simulink library "mssSimulink"  (R2024a)
settings: Solver=ode45  StartTime=0.0  StopTime=10.0  RelTol=1e-3
undefined symbols (not defined in the file): ABC, CN_data, CX_data, CY_data, D, G, Hoerner, K_supply, kt2ms, MA, magnitude, MRB, pathlength, RAO_Amp, RAO_Dir, RAO_Freq, RAO_Phase, RAO_Vel, RAO_yaw_back, RAO_yaw_quant, RAO_yaw_quantization_flag, rho_a, slcm, T_supply, table, vessel, vesselABC
libraries: $bdroot x99, simulink x13
(part 8 of 9)

== system mssSimulink/Guidance/Waypoint guidance block/vs_calculations/vs_theta_calc ==
  xd_theta : Inport
  xd_theta_2 : Inport  Port=2
  yd_theta : Inport  Port=3
  yd_theta_2 : Inport  Port=4
  ud : Inport  Port=5
  Fcn1 : Fcn  Expr=u^(3/2)
  Gain1 : Gain  Gain=-1  SaturateOnIntegerOverflow=on  OutDataTypeStr=Inherit: Same as input  ParamDataTypeStr=Inherit: Same as input
  Math Function2 : Math  Operator=square  SignedPower=on
  Math Function3 : Math  Operator=square  SignedPower=on
  Product4 : Product  InputSameDT=on  SaturateOnIntegerOverflow=on  OutDataTypeStr=Inherit: Same as first input
  Product5 : Product  InputSameDT=on  SaturateOnIntegerOverflow=on  OutDataTypeStr=Inherit: Same as first input
  Product6 : Product  Inputs=/*  InputSameDT=on  SaturateOnIntegerOverflow=on  OutDataTypeStr=Inherit: Same as first input
  Product7 : Product  InputSameDT=on  SaturateOnIntegerOverflow=on  OutDataTypeStr=Inherit: Same as first input
  Sum2 : Sum  Inputs=|++  InputSameDT=on  SaturateOnIntegerOverflow=on  OutDataTypeStr=Inherit: Same as first input
  Sum3 : Sum  Inputs=|++  InputSameDT=on  SaturateOnIntegerOverflow=on  OutDataTypeStr=Inherit: Same as first input
  vs_theta : Outport  VectorParamsAs1DForOutWhenUnconnected=off
  wires:
  xd_theta/1 -> Math Function2/1, Product4/1
  yd_theta/1 -> Math Function3/1, Product5/1
  Math Function2/1 -> Sum2/1
  Math Function3/1 -> Sum2/2
  Sum2/1 -> Fcn1/1
  xd_theta_2/1 -> Product4/2
  yd_theta_2/1 -> Product5/2
  Product4/1 -> Sum3/1
  Product5/1 -> Sum3/2
  Fcn1/1 -> Product6/1
  Sum3/1 -> Product6/2
  Product6/1 -> Gain1/1
  Gain1/1 -> Product7/1
  ud/1 -> Product7/2
  Product7/1 -> vs_theta/1

== system mssSimulink/Hydrodynamics/6-DOF maneuvering model (unified model with fluid memory)/Model Info1/EmptySubsystem ==

== system mssSimulink/Hydrodynamics/Cross-flow drag and surge resistance/Cross-flow drag trapezoidal integration/multiply with 0.5 ==
  In1 : Inport
  Action Port : ActionPort  InitializeStates=reset
  Gain : Gain  Gain=0.5
  Out1 : Outport
  wires:
  In1/1 -> Gain/1
  Gain/1 -> Out1/1

== system mssSimulink/Hydrodynamics/Cross-flow drag and surge resistance/Cross-flow drag trapezoidal integration/multiply with 1 ==
  In1 : Inport
  Action Port : ActionPort  InitializeStates=reset
  Out1 : Outport
  wires:
  In1/1 -> Out1/1

== system mssSimulink/Hydrodynamics/WD for heading1/Wave component loop/WD RAO tables ==
  beta : Inport
  w : Inport  Port=2
  U : Inport  Port=3
  Constant : Constant  Value=0
  Lookup Table (n-D) Wavedrift 1 : Lookup_n-D  NumberOfTableDimensions=3  BreakpointsForDimension1=WD_Freq  BreakpointsForDimension2=vessel.headings  BreakpointsForDimension3=RAO_Vel  IndexSearchMethod=Linear search  BeginIndexSearchUsingPreviousIndexResult=on  Table=WD_Amp{1}  ExtrapMethod=Clip  DiagnosticForOutOfRangeInput=Warning  InternalRulePriority=Speed  RndMeth=Simplest
      settings: InputPortMap=u0,u1,u2
  Lookup Table (n-D) Wavedrift 2 : Lookup_n-D  NumberOfTableDimensions=3  BreakpointsForDimension1=WD_Freq  BreakpointsForDimension2=vessel.headings  BreakpointsForDimension3=RAO_Vel  IndexSearchMethod=Linear search  BeginIndexSearchUsingPreviousIndexResult=on  Table=WD_Amp{2}  ExtrapMethod=Clip  DiagnosticForOutOfRangeInput=Warning  InternalRulePriority=Speed  RndMeth=Simplest
      settings: InputPortMap=u0,u1,u2
  Lookup Table (n-D) Wavedrift 3 : Lookup_n-D  NumberOfTableDimensions=3  BreakpointsForDimension1=WD_Freq  BreakpointsForDimension2=vessel.headings  BreakpointsForDimension3=RAO_Vel  IndexSearchMethod=Linear search  BeginIndexSearchUsingPreviousIndexResult=on  Table=WD_Amp{3}  ExtrapMethod=Clip  DiagnosticForOutOfRangeInput=Warning  InternalRulePriority=Speed  RndMeth=Simplest
      settings: InputPortMap=u0,u1,u2
  Mux1 : Mux  Inputs=6
  amp : Outport
  wires:
  Mux1/1 -> amp/1
  Lookup Table (n-D) Wavedrift 3/1 -> Mux1/6
  Lookup Table (n-D) Wavedrift 2/1 -> Mux1/2
  Lookup Table (n-D) Wavedrift 1/1 -> Mux1/1
  U/1 -> Lookup Table (n-D) Wavedrift 2/3, Lookup Table (n-D) Wavedrift 3/3, Lookup Table (n-D) Wavedrift 1/3
  beta/1 -> Lookup Table (n-D) Wavedrift 2/2, Lookup Table (n-D) Wavedrift 3/2, Lookup Table (n-D) Wavedrift 1/2
  Constant/1 -> Mux1/3, Mux1/4, Mux1/5
  w/1 -> Lookup Table (n-D) Wavedrift 2/1, Lookup Table (n-D) Wavedrift 3/1, Lookup Table (n-D) Wavedrift 1/1

== system mssSimulink/Hydrodynamics/WD for heading1/Wave component loop/[-pi pi] to [0 2pi] ==
  note: x
  x [-pi pi] : Inport
  Constant : Constant  Value=2*pi
  Constant1 : Constant  Value=0
  Sign : Signum
  Sum : Sum  Inputs=|++  SaturateOnIntegerOverflow=on
  Switch : Switch  SaturateOnIntegerOverflow=off  InputSameDT=off
  0<y<2pi : Outport
  wires:
  x [-pi pi]/1 -> Sign/1, Sum/2
  Switch/1 -> Sum/1
  Sum/1 -> 0<y<2pi/1
  Sign/1 -> Switch/2
  Constant/1 -> Switch/3
  Constant1/1 -> Switch/1

== system mssSimulink/Hydrodynamics/Wave loads (U>0)/Wave loads U = U1/psi1 ==
  k : Inport
  0 or 1 : Inport  Port=2
  Gain1 : Gain  Gain=20
  Gain2 : Gain  Gain=10
  Product : Product  RndMeth=Zero
  Sum7 : Sum  Inputs=-+|
  Sum8 : Sum  Inputs=++|
  const : Constant  Value=18
  psi : Outport
  wires:
  0 or 1/1 -> Product/2
  Sum8/1 -> psi/1
  k/1 -> Gain2/1, Sum7/1
  Gain2/1 -> Sum8/1
  Product/1 -> Sum8/2
  Gain1/1 -> Product/1
  Sum7/1 -> Gain1/1
  const/1 -> Sum7/2

== system mssSimulink/Hydrodynamics/Wave loads (U>0)/Wave loads U = U1/psi2 ==
  k : Inport
  0 or 1 : Inport  Port=2
  Gain1 : Gain  Gain=20
  Gain2 : Gain  Gain=10
  Product : Product  RndMeth=Zero
  Sum7 : Sum  Inputs=-+|
  Sum8 : Sum  Inputs=++|
  const : Constant  Value=18
  psi : Outport
  wires:
  0 or 1/1 -> Product/2
  Sum8/1 -> psi/1
  k/1 -> Gain2/1, Sum7/1
  Gain2/1 -> Sum8/1
  Product/1 -> Sum8/2
  Gain1/1 -> Product/1
  Sum7/1 -> Gain1/1
  const/1 -> Sum7/2

== system mssSimulink/Hydrodynamics/Wave loads (U>0)/Wave loads U = U2/Wave loads for heading1 ==
  eta : Inport
  psi : Inport  Port=2
  psi_wave : Inport  Port=3
  wavenum : Inport  Port=4
  Omega : Inport  Port=5
  Phase : Inport  Port=6
  Zeta_a : Inport  Port=7
  U_idx : Inport  Port=8
  Clock : Clock
  "Position phase " : $bdroot/Modelling/Environmental Loads/Utilities/Position phase
  Product1 : Product  Inputs=**  SaturateOnIntegerOverflow=on  OutDataTypeStr=Inherit: Same as first input
  Sum : Sum  Inputs=-++  SaturateOnIntegerOverflow=on
  Sum1 : Sum  Inputs=-+|
  Wave component loop : Subsystem  TreatAsAtomicUnit=on
  Width : Width  DataType=int32
  tau_WF : Outport
  tau_WD : Outport  Port=2
  wires:
  psi/1 -> Sum1/1  "psi"
  U_idx/1 -> Wave component loop/6(U_idx)
  Wave component loop/2(tau_WD) -> tau_WD/1
  Sum1/1 -> Wave component loop/2(Psi_r)
  Zeta_a/1 -> Wave component loop/5(Zeta_a)
  Phase/1 -> Sum/3
  Omega/1 -> Width/1, Wave component loop/3(Omega), Product1/1
  wavenum/1 -> "Position phase "/2
  psi_wave/1 -> Sum1/2, "Position phase "/1
  eta/1 -> "Position phase "/3
  Wave component loop/1(tau_WF) -> tau_WF/1
  Product1/1 -> Sum/2
  Clock/1 -> Product1/2
  Sum/1 -> Wave component loop/4(Phase_tot)  "Phase_tot"
  Width/1 -> Wave component loop/1(number of iterations)
  "Position phase "/1 -> Sum/1

== system mssSimulink/Hydrodynamics/Wave loads (U>0)/Wave loads U = U2/Wave loads for heading2 ==
  eta : Inport
  psi : Inport  Port=2
  psi_wave : Inport  Port=3
  wavenum : Inport  Port=4
  Omega : Inport  Port=5
  Phase : Inport  Port=6
  Zeta_a : Inport  Port=7
  U : Inport  Port=8
  Clock : Clock
  "Position phase " : $bdroot/Modelling/Environmental Loads/Utilities/Position phase
  Product1 : Product  Inputs=**  SaturateOnIntegerOverflow=on  OutDataTypeStr=Inherit: Same as first input
  Sum : Sum  Inputs=-++  SaturateOnIntegerOverflow=on
  Sum1 : Sum  Inputs=-+|
  Wave component loop : Subsystem  TreatAsAtomicUnit=on
  Width : Width  DataType=int32
  tau_WF : Outport
  tau_WD : Outport  Port=2
  wires:
  psi/1 -> Sum1/1  "psi"
  U/1 -> Wave component loop/6(U)
  Wave component loop/2(tau_WD) -> tau_WD/1
  Sum1/1 -> Wave component loop/2(Psi_r)
  Zeta_a/1 -> Wave component loop/5(Zeta_a)
  Phase/1 -> Sum/3
  Omega/1 -> Width/1, Wave component loop/3(Omega), Product1/1
  wavenum/1 -> "Position phase "/2
  psi_wave/1 -> Sum1/2, "Position phase "/1
  eta/1 -> "Position phase "/3
  Wave component loop/1(tau_WF) -> tau_WF/1
  Product1/1 -> Sum/2
  Clock/1 -> Product1/2
  Sum/1 -> Wave component loop/4(Phase_tot)  "Phase_tot"
  Width/1 -> Wave component loop/1(number of iterations)
  "Position phase "/1 -> Sum/1

== system mssSimulink/Hydrodynamics/Wave loads (U>0)/Wave loads U = U2/psi1 ==
  k : Inport
  0 or 1 : Inport  Port=2
  Gain1 : Gain  Gain=20
  Gain2 : Gain  Gain=10
  Product : Product  RndMeth=Zero
  Sum7 : Sum  Inputs=-+|
  Sum8 : Sum  Inputs=++|
  const : Constant  Value=18
  psi : Outport
  wires:
  0 or 1/1 -> Product/2
  Sum8/1 -> psi/1
  k/1 -> Gain2/1, Sum7/1
  Gain2/1 -> Sum8/1
  Product/1 -> Sum8/2
  Gain1/1 -> Product/1
  Sum7/1 -> Gain1/1
  const/1 -> Sum7/2

== system mssSimulink/Hydrodynamics/Wave loads (U>0)/Wave loads U = U2/psi2 ==
  k : Inport
  0 or 1 : Inport  Port=2
  Gain1 : Gain  Gain=20
  Gain2 : Gain  Gain=10
  Product : Product  RndMeth=Zero
  Sum7 : Sum  Inputs=-+|
  Sum8 : Sum  Inputs=++|
  const : Constant  Value=18
  psi : Outport
  wires:
  0 or 1/1 -> Product/2
  Sum8/1 -> psi/1
  k/1 -> Gain2/1, Sum7/1
  Gain2/1 -> Sum8/1
  Product/1 -> Sum8/2
  Gain1/1 -> Product/1
  Sum7/1 -> Gain1/1
  const/1 -> Sum7/2

== system mssSimulink/Hydrodynamics/Wave loads for heading1/Wave component loop/Force RAO tables ==
  beta : Inport
  w : Inport  Port=2
  U : Inport  Port=3
  Lookup Table (n-D) Amp1 : Lookup_n-D  NumberOfTableDimensions=3  BreakpointsForDimension1=ForceRAO_Freq  BreakpointsForDimension2=vessel.headings  BreakpointsForDimension3=RAO_Vel  IndexSearchMethod=Linear search  BeginIndexSearchUsingPreviousIndexResult=on  Table=ForceRAO_Amp{1}  ExtrapMethod=Clip  DiagnosticForOutOfRangeInput=Warning  InternalRulePriority=Speed  RndMeth=Simplest
      settings: InputPortMap=u0,u1,u2
  Lookup Table (n-D) Amp2 : Lookup_n-D  NumberOfTableDimensions=3  BreakpointsForDimension1=ForceRAO_Freq  BreakpointsForDimension2=vessel.headings  BreakpointsForDimension3=RAO_Vel  IndexSearchMethod=Linear search  BeginIndexSearchUsingPreviousIndexResult=on  Table=ForceRAO_Amp{2}  ExtrapMethod=Clip  DiagnosticForOutOfRangeInput=Warning  InternalRulePriority=Speed  RndMeth=Simplest
      settings: InputPortMap=u0,u1,u2
  Lookup Table (n-D) Amp3 : Lookup_n-D  NumberOfTableDimensions=3  BreakpointsForDimension1=ForceRAO_Freq  BreakpointsForDimension2=vessel.headings  BreakpointsForDimension3=RAO_Vel  IndexSearchMethod=Linear search  BeginIndexSearchUsingPreviousIndexResult=on  Table=ForceRAO_Amp{3}  ExtrapMethod=Clip  DiagnosticForOutOfRangeInput=Warning  InternalRulePriority=Speed  RndMeth=Simplest
      settings: InputPortMap=u0,u1,u2
  Lookup Table (n-D) Amp4 : Lookup_n-D  NumberOfTableDimensions=3  BreakpointsForDimension1=ForceRAO_Freq  BreakpointsForDimension2=vessel.headings  BreakpointsForDimension3=RAO_Vel  IndexSearchMethod=Linear search  BeginIndexSearchUsingPreviousIndexResult=on  Table=ForceRAO_Amp{4}  ExtrapMethod=Clip  DiagnosticForOutOfRangeInput=Warning  InternalRulePriority=Speed  RndMeth=Simplest
      settings: InputPortMap=u0,u1,u2
  Lookup Table (n-D) Amp5 : Lookup_n-D  NumberOfTableDimensions=3  BreakpointsForDimension1=ForceRAO_Freq  BreakpointsForDimension2=vessel.headings  BreakpointsForDimension3=RAO_Vel  IndexSearchMethod=Linear search  BeginIndexSearchUsingPreviousIndexResult=on  Table=ForceRAO_Amp{5}  ExtrapMethod=Clip  DiagnosticForOutOfRangeInput=Warning  InternalRulePriority=Speed  RndMeth=Simplest
      settings: InputPortMap=u0,u1,u2
  Lookup Table (n-D) Amp6 : Lookup_n-D  NumberOfTableDimensions=3  BreakpointsForDimension1=ForceRAO_Freq  BreakpointsForDimension2=vessel.headings  BreakpointsForDimension3=RAO_Vel  IndexSearchMethod=Linear search  BeginIndexSearchUsingPreviousIndexResult=on  Table=ForceRAO_Amp{6}  ExtrapMethod=Clip  DiagnosticForOutOfRangeInput=Warning  InternalRulePriority=Speed  RndMeth=Simplest
      settings: InputPortMap=u0,u1,u2
  Lookup Table (n-D) Phase : Lookup_n-D  NumberOfTableDimensions=3  BreakpointsForDimension1=ForceRAO_Freq  BreakpointsForDimension2=vessel.headings  BreakpointsForDimension3=RAO_Vel  IndexSearchMethod=Linear search  BeginIndexSearchUsingPreviousIndexResult=on  Table=ForceRAO_Phase{3}  ExtrapMethod=Clip  DiagnosticForOutOfRangeInput=Warning  InternalRulePriority=Speed  RndMeth=Simplest
      settings: InputPortMap=u0,u1,u2
  Lookup Table (n-D) Phase1 : Lookup_n-D  NumberOfTableDimensions=3  BreakpointsForDimension1=ForceRAO_Freq  BreakpointsForDimension2=vessel.headings  BreakpointsForDimension3=RAO_Vel  IndexSearchMethod=Linear search  BeginIndexSearchUsingPreviousIndexResult=on  Table=ForceRAO_Phase{1}  ExtrapMethod=Clip  DiagnosticForOutOfRangeInput=Warning  InternalRulePriority=Speed  RndMeth=Simplest
      settings: InputPortMap=u0,u1,u2
  Lookup Table (n-D) Phase2 : Lookup_n-D  NumberOfTableDimensions=3  BreakpointsForDimension1=ForceRAO_Freq  BreakpointsForDimension2=vessel.headings  BreakpointsForDimension3=RAO_Vel  IndexSearchMethod=Linear search  BeginIndexSearchUsingPreviousIndexResult=on  Table=ForceRAO_Phase{2}  ExtrapMethod=Clip  DiagnosticForOutOfRangeInput=Warning  InternalRulePriority=Speed  RndMeth=Simplest
      settings: InputPortMap=u0,u1,u2
  Lookup Table (n-D) Phase4 : Lookup_n-D  NumberOfTableDimensions=3  BreakpointsForDimension1=ForceRAO_Freq  BreakpointsForDimension2=vessel.headings  BreakpointsForDimension3=RAO_Vel  IndexSearchMethod=Linear search  BeginIndexSearchUsingPreviousIndexResult=on  Table=ForceRAO_Phase{4}  ExtrapMethod=Clip  DiagnosticForOutOfRangeInput=Warning  InternalRulePriority=Speed  RndMeth=Simplest
      settings: InputPortMap=u0,u1,u2
  Lookup Table (n-D) Phase5 : Lookup_n-D  NumberOfTableDimensions=3  BreakpointsForDimension1=ForceRAO_Freq  BreakpointsForDimension2=vessel.headings  BreakpointsForDimension3=RAO_Vel  IndexSearchMethod=Linear search  BeginIndexSearchUsingPreviousIndexResult=on  Table=ForceRAO_Phase{5}  ExtrapMethod=Clip  DiagnosticForOutOfRangeInput=Warning  InternalRulePriority=Speed  RndMeth=Simplest
      settings: InputPortMap=u0,u1,u2
  Lookup Table (n-D) Phase6 : Lookup_n-D  NumberOfTableDimensions=3  BreakpointsForDimension1=ForceRAO_Freq  BreakpointsForDimension2=vessel.headings  BreakpointsForDimension3=RAO_Vel  IndexSearchMethod=Linear search  BeginIndexSearchUsingPreviousIndexResult=on  Table=ForceRAO_Phase{6}  ExtrapMethod=Clip  DiagnosticForOutOfRangeInput=Warning  InternalRulePriority=Speed  RndMeth=Simplest
      settings: InputPortMap=u0,u1,u2
  Mux1 : Mux  Inputs=6
  Mux2 : Mux  Inputs=6
  amp : Outport
  phase : Outport  Port=2
  wires:
  w/1 -> Lookup Table (n-D) Amp1/1, Lookup Table (n-D) Amp2/1, Lookup Table (n-D) Amp3/1, Lookup Table (n-D) Amp4/1, Lookup Table (n-D) Amp5/1, Lookup Table (n-D) Amp6/1, Lookup Table (n-D) Phase1/1, Lookup Table (n-D) Phase2/1, Lookup Table (n-D) Phase/1, Lookup Table (n-D) Phase4/1, Lookup Table (n-D) Phase6/1, Lookup Table (n-D) Phase5/1
  Lookup Table (n-D) Phase5/1 -> Mux2/5
  Lookup Table (n-D) Phase/1 -> Mux2/3
  Lookup Table (n-D) Phase1/1 -> Mux2/1
  beta/1 -> Lookup Table (n-D) Amp1/2, Lookup Table (n-D) Amp2/2, Lookup Table (n-D) Amp3/2, Lookup Table (n-D) Amp4/2, Lookup Table (n-D) Amp5/2, Lookup Table (n-D) Amp6/2, Lookup Table (n-D) Phase1/2, Lookup Table (n-D) Phase2/2, Lookup Table (n-D) Phase/2, Lookup Table (n-D) Phase4/2, Lookup Table (n-D) Phase6/2, Lookup Table (n-D) Phase5/2
  Lookup Table (n-D) Phase4/1 -> Mux2/4
  Lookup Table (n-D) Phase2/1 -> Mux2/2
  Lookup Table (n-D) Phase6/1 -> Mux2/6
  Lookup Table (n-D) Amp4/1 -> Mux1/4
  U/1 -> Lookup Table (n-D) Amp1/3, Lookup Table (n-D) Amp2/3, Lookup Table (n-D) Amp3/3, Lookup Table (n-D) Amp4/3, Lookup Table (n-D) Amp5/3, Lookup Table (n-D) Amp6/3, Lookup Table (n-D) Phase1/3, Lookup Table (n-D) Phase2/3, Lookup Table (n-D) Phase/3, Lookup Table (n-D) Phase4/3, Lookup Table (n-D) Phase6/3, Lookup Table (n-D) Phase5/3
  Lookup Table (n-D) Amp1/1 -> Mux1/1
  Lookup Table (n-D) Amp3/1 -> Mux1/3
  Lookup Table (n-D) Amp5/1 -> Mux1/5
  Lookup Table (n-D) Amp2/1 -> Mux1/2
  Lookup Table (n-D) Amp6/1 -> Mux1/6
  Mux2/1 -> phase/1
  Mux1/1 -> amp/1

== system mssSimulink/Hydrodynamics/Wave loads for heading1/Wave component loop/WD RAO tables ==
  beta : Inport
  w : Inport  Port=2
  U : Inport  Port=3
  Constant : Constant  Value=0
  Lookup Table (n-D) Wavedrift 1 : Lookup_n-D  NumberOfTableDimensions=3  BreakpointsForDimension1=WD_Freq  BreakpointsForDimension2=vessel.headings  BreakpointsForDimension3=RAO_Vel  IndexSearchMethod=Linear search  BeginIndexSearchUsingPreviousIndexResult=on  Table=WD_Amp{1}  ExtrapMethod=Clip  DiagnosticForOutOfRangeInput=Warning  InternalRulePriority=Speed  RndMeth=Simplest
      settings: InputPortMap=u0,u1,u2
  Lookup Table (n-D) Wavedrift 2 : Lookup_n-D  NumberOfTableDimensions=3  BreakpointsForDimension1=WD_Freq  BreakpointsForDimension2=vessel.headings  BreakpointsForDimension3=RAO_Vel  IndexSearchMethod=Linear search  BeginIndexSearchUsingPreviousIndexResult=on  Table=WD_Amp{2}  ExtrapMethod=Clip  DiagnosticForOutOfRangeInput=Warning  InternalRulePriority=Speed  RndMeth=Simplest
      settings: InputPortMap=u0,u1,u2
  Lookup Table (n-D) Wavedrift 3 : Lookup_n-D  NumberOfTableDimensions=3  BreakpointsForDimension1=WD_Freq  BreakpointsForDimension2=vessel.headings  BreakpointsForDimension3=RAO_Vel  IndexSearchMethod=Linear search  BeginIndexSearchUsingPreviousIndexResult=on  Table=WD_Amp{3}  ExtrapMethod=Clip  DiagnosticForOutOfRangeInput=Warning  InternalRulePriority=Speed  RndMeth=Simplest
      settings: InputPortMap=u0,u1,u2
  Mux1 : Mux  Inputs=6
  amp : Outport
  wires:
  w/1 -> Lookup Table (n-D) Wavedrift 1/1, Lookup Table (n-D) Wavedrift 3/1, Lookup Table (n-D) Wavedrift 2/1
  Constant/1 -> Mux1/5, Mux1/4, Mux1/3
  beta/1 -> Lookup Table (n-D) Wavedrift 1/2, Lookup Table (n-D) Wavedrift 3/2, Lookup Table (n-D) Wavedrift 2/2
  U/1 -> Lookup Table (n-D) Wavedrift 1/3, Lookup Table (n-D) Wavedrift 3/3, Lookup Table (n-D) Wavedrift 2/3
  Lookup Table (n-D) Wavedrift 1/1 -> Mux1/1
  Lookup Table (n-D) Wavedrift 2/1 -> Mux1/2
  Lookup Table (n-D) Wavedrift 3/1 -> Mux1/6
  Mux1/1 -> amp/1

== system mssSimulink/Hydrodynamics/Wave loads for heading1/Wave component loop/[-pi pi] to [0 2pi] ==
  note: x
  x [-pi pi] : Inport
  Constant : Constant  Value=2*pi
  Constant1 : Constant  Value=0
  Sign : Signum
  Sum : Sum  Inputs=|++  SaturateOnIntegerOverflow=on
  Switch : Switch  SaturateOnIntegerOverflow=off  InputSameDT=off
  0<y<2pi : Outport
  wires:
  Constant1/1 -> Switch/1
  Constant/1 -> Switch/3
  Sign/1 -> Switch/2
  Sum/1 -> 0<y<2pi/1
  Switch/1 -> Sum/1
  x [-pi pi]/1 -> Sum/2, Sign/1

== system mssSimulink/Modelling/Environmental Loads/Force RAO/Wave component loop ==
  number of iterations : Inport
  Psi_r : Inport  Port=2
  Omega : Inport  Port=3
  Phase_tot : Inport  Port=4
  Zeta_a : Inport  Port=5
  U : Inport  Port=6
  "                " : Trigonometry
  "                1" : Trigonometry  Operator=cos
  For Iterator : ForIterator  ResetStates=reset  IterationSource=external  IterationVariableDataType=double
  Memory1 : Memory  InitialCondition=[0 0 0 0 0 0]'  InheritSampleTime=on
  Memory2 : Memory  InitialCondition=[0 0 0 0 0 0]'  InheritSampleTime=on
  Product1 : Product  SaturateOnIntegerOverflow=on  OutDataTypeStr=Inherit: Same as first input
  Product3 : Product  Inputs=3  SaturateOnIntegerOverflow=on  OutDataTypeStr=Inherit: Same as first input
  Product4 : Product  SaturateOnIntegerOverflow=on  OutDataTypeStr=Inherit: Same as first input
  "RAO tables " : $bdroot/Modelling/Environmental Loads/Utilities/RAO tables  RAO_Freq=RAO_Freq  RAO_Dir=RAO_Dir  RAO_Vel=RAO_Vel  RAO_Amp=RAO_Amp  RAO_Phase=RAO_Phase
  Selector{2..5} (4 alike) : Selector  IndexOptions=Index vector (port)  Indices=[1 3]  OutputSizes=1
  Sum1 : Sum  Inputs=++|  SaturateOnIntegerOverflow=on
  Sum4 : Sum  Inputs=++|  SaturateOnIntegerOverflow=on
  Sum5 : Sum  Inputs=++|  SaturateOnIntegerOverflow=on
  Tau WF : Outport  VectorParamsAs1DForOutWhenUnconnected=off
  Tau rate : Outport  Port=2  VectorParamsAs1DForOutWhenUnconnected=off
  wires:
  "                1"/1 -> Product3/1
  Sum1/1 -> Memory1/1, Tau rate/1
  Memory1/1 -> Sum1/2
  Product3/1 -> Sum1/1
  Product4/1 -> Product3/2, Product1/2
  "                "/1 -> Product1/1
  Selector3/1 -> "RAO tables "/1  "psi_r"
  Selector2/1 -> Product3/3, "RAO tables "/2  "omega"
  Selector5/1 -> Sum5/2  "phase"
  Product1/1 -> Sum4/1
  Memory2/1 -> Sum4/2
  Sum4/1 -> Tau WF/1, Memory2/1
  number of iterations/1 -> For Iterator/1
  Omega/1 -> Selector2/1
  For Iterator/1 -> Selector4/2, Selector5/2, Selector2/2, Selector3/2  "i=1:N"
  Psi_r/1 -> Selector3/1
  U/1 -> "RAO tables "/3
  "RAO tables "/1 -> Product4/1
  "RAO tables "/2 -> Sum5/1
  Phase_tot/1 -> Selector5/1
  Zeta_a/1 -> Selector4/1
  Sum5/1 -> "                1"/1, "                "/1
  Selector4/1 -> Product4/2  "zeta_a"

== system mssSimulink/Modelling/Environmental Loads/Motion RAO/6DOF rotation matrix in yaw ==
  psi : Inport
  V : Inport  Port=2
  Mux1 : Mux  Inputs=2
  Rotation matrix in yaw : $bdroot/Modelling/Kinematics/Rotation matrix in yaw 
  Selector : Selector  InputPortWidth=6  IndexOptions=Index vector (dialog)  Indices=[4 5 6]  OutputSizes=1
  Selector2 : Selector  InputPortWidth=6  IndexOptions=Index vector (dialog)  Indices=[1 2 3]  OutputSizes=1
  R(psi)*V : Outport  VectorParamsAs1DForOutWhenUnconnected=off
  wires:
  Rotation matrix in yaw/1 -> Mux1/1
  V/1 -> Selector/1, Selector2/1
  psi/1 -> Rotation matrix in yaw/1
  Selector2/1 -> Rotation matrix in yaw/2
  Mux1/1 -> R(psi)*V/1
  Selector/1 -> Mux1/2

== system mssSimulink/Modelling/Environmental Loads/Motion RAO/Output smoothing ==
  eta_h WF : Inport
  "nu WF " : Inport  Port=2
  "nu_dot WF " : Inport  Port=3
  nu_dot rate : Inport  Port=4
  Output smoothing flag : Constant  Value=RAO_smoothing_flag
  "Signal smoothing 1 " : $bdroot/Modelling/Environmental Loads/Utilities/Signal smoothing
  Signal smoothing 2 : $bdroot/Modelling/Environmental Loads/Utilities/Signal smoothing
  Signal smoothing 3 : $bdroot/Modelling/Environmental Loads/Utilities/Signal smoothing
  Switch1 : Switch  Threshold=0.5  SaturateOnIntegerOverflow=off  InputSameDT=off
  Switch2 : Switch  Threshold=0.5  SaturateOnIntegerOverflow=off  InputSameDT=off
  Switch3 : Switch  Threshold=0.5  SaturateOnIntegerOverflow=off  InputSameDT=off
  "eta_h WF " : Outport  VectorParamsAs1DForOutWhenUnconnected=off
  nu WF : Outport  Port=2  VectorParamsAs1DForOutWhenUnconnected=off
  nu_dot WF : Outport  Port=3  VectorParamsAs1DForOutWhenUnconnected=off
  wires:
  Switch1/1 -> nu WF/1
  Switch3/1 -> nu_dot WF/1
  nu_dot rate/1 -> Signal smoothing 3/2
  Signal smoothing 3/1 -> Switch3/1
  "nu_dot WF "/1 -> Switch3/3, Signal smoothing 2/2, Signal smoothing 3/1
  Switch2/1 -> "eta_h WF "/1
  Signal smoothing 2/1 -> Switch1/1
  "nu WF "/1 -> Switch1/3, "Signal smoothing 1 "/2, Signal smoothing 2/1
  eta_h WF/1 -> Switch2/3, "Signal smoothing 1 "/1
  "Signal smoothing 1 "/1 -> Switch2/1
  Output smoothing flag/1 -> Switch3/2, Switch1/2, Switch2/2

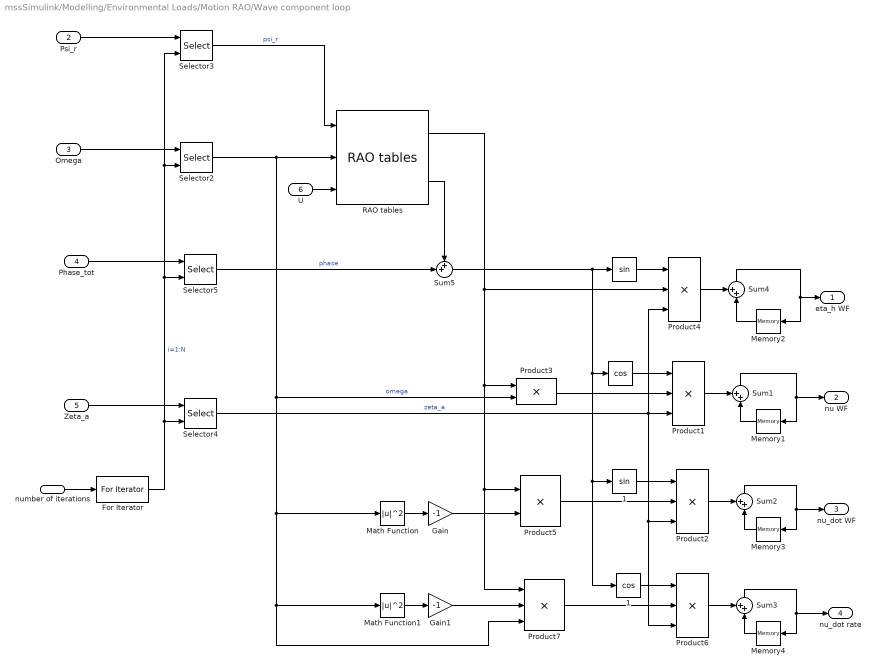
== system mssSimulink/Modelling/Environmental Loads/Motion RAO/Wave component loop ==
  number of iterations : Inport
  Psi_r : Inport  Port=2
  Omega : Inport  Port=3
  Phase_tot : Inport  Port=4
  Zeta_a : Inport  Port=5
  U : Inport  Port=6
  "              " : Trigonometry  Operator=cos
  "                " : Trigonometry
  "                1" : Trigonometry
  "              1" : Trigonometry  Operator=cos
  For Iterator : ForIterator  ResetStates=reset  IterationSource=external  IterationVariableDataType=double
  Gain : Gain  Gain=-1  SaturateOnIntegerOverflow=on  OutDataTypeStr=Inherit: Same as input  ParamDataTypeStr=Inherit: Same as input
  Gain1 : Gain  Gain=-1  SaturateOnIntegerOverflow=on  OutDataTypeStr=Inherit: Same as input  ParamDataTypeStr=Inherit: Same as input
  Math Function : Math  Operator=magnitude^2  SignedPower=on
  Math Function1 : Math  Operator=magnitude^2  SignedPower=on
  Memory{1..4} (4 alike) : Memory  InitialCondition=[0 0 0 0 0 0]'  InheritSampleTime=on
  Product{1..2,4,6} (4 alike) : Product  Inputs=3  SaturateOnIntegerOverflow=on  OutDataTypeStr=Inherit: Same as first input
  Product3 : Product  Inputs=**  SaturateOnIntegerOverflow=on  OutDataTypeStr=Inherit: Same as first input
  Product5 : Product  Inputs=**  SaturateOnIntegerOverflow=on  OutDataTypeStr=Inherit: Same as first input
  Product7 : Product  Inputs=***  SaturateOnIntegerOverflow=on  OutDataTypeStr=Inherit: Same as first input
  "RAO tables " : $bdroot/Modelling/Environmental Loads/Utilities/RAO tables  RAO_Freq=RAO_Freq  RAO_Dir=RAO_Dir  RAO_Vel=RAO_Vel  RAO_Amp=RAO_Amp  RAO_Phase=RAO_Phase
  Selector{2..5} (4 alike) : Selector  IndexOptions=Index vector (port)  Indices=[1 3]  OutputSizes=1
  Sum{1..5} (5 alike) : Sum  Inputs=++|  SaturateOnIntegerOverflow=on
  eta_h WF : Outport  VectorParamsAs1DForOutWhenUnconnected=off
  nu WF : Outport  Port=2  VectorParamsAs1DForOutWhenUnconnected=off
  nu_dot WF : Outport  Port=3  VectorParamsAs1DForOutWhenUnconnected=off
  nu_dot rate : Outport  Port=4  VectorParamsAs1DForOutWhenUnconnected=off
  wires:
  Product7/1 -> Product6/2
  "              1"/1 -> Product6/1
  Math Function1/1 -> Gain1/1
  Gain1/1 -> Product7/2
  Memory4/1 -> Sum3/2
  Product6/1 -> Sum3/1
  Sum3/1 -> Memory4/1, nu_dot rate/1
  Selector3/1 -> "RAO tables "/1  "psi_r"
  Selector2/1 -> Product7/3, Math Function1/1, Math Function/1, Product3/2, "RAO tables "/2  "omega"
  Selector5/1 -> Sum5/2  "phase"
  Product4/1 -> Sum4/1
  Memory2/1 -> Sum4/2
  Sum4/1 -> eta_h WF/1, Memory2/1
  number of iterations/1 -> For Iterator/1
  Omega/1 -> Selector2/1
  For Iterator/1 -> Selector3/2, Selector2/2, Selector5/2, Selector4/2  "i=1:N"
  Psi_r/1 -> Selector3/1
  U/1 -> "RAO tables "/3
  "RAO tables "/1 -> Product4/2, Product7/1, Product5/1, Product3/1
  "RAO tables "/2 -> Sum5/1
  Phase_tot/1 -> Selector5/1
  Zeta_a/1 -> Selector4/1
  Sum5/1 -> "                "/1, "              1"/1, "                1"/1, "              "/1
  "                "/1 -> Product4/1
  Selector4/1 -> Product6/3, Product2/3, Product1/3, Product4/3  "zeta_a"
  "              "/1 -> Product1/1
  Memory1/1 -> Sum1/2
  Sum1/1 -> nu WF/1, Memory1/1
  Product1/1 -> Sum1/1
  Memory3/1 -> Sum2/2
  Product2/1 -> Sum2/1
  Sum2/1 -> nu_dot WF/1, Memory3/1
  "                1"/1 -> Product2/1
  Math Function/1 -> Gain/1
  Gain/1 -> Product5/2
  Product5/1 -> Product2/2
  Product3/1 -> Product1/2

== system mssSimulink/Modelling/Environmental Loads/Utilities/Position phase ==
  psi wave : Inport
  wavenum : Inport  Port=2
  eta LF : Inport  Port=3
  Product2 : Product  Inputs=**  SaturateOnIntegerOverflow=on  OutDataTypeStr=Inherit: Same as first input
  Product6 : Product  Inputs=**  SaturateOnIntegerOverflow=on  OutDataTypeStr=Inherit: Same as first input
  Product7 : Product  Inputs=**  SaturateOnIntegerOverflow=on  OutDataTypeStr=Inherit: Same as first input
  Sum5 : Sum  SaturateOnIntegerOverflow=on
  cos : Trigonometry  Operator=cos
  sin : Trigonometry
  x-position : Selector  IndexOptions=Index vector (dialog)  Indices=1  OutputSizes=1
  y-position : Selector  InputPortWidth=6  IndexOptions=Index vector (dialog)  Indices=2  OutputSizes=1
  pos phase : Outport  VectorParamsAs1DForOutWhenUnconnected=off
  wires:
  wavenum/1 -> Product7/2
  Product7/1 -> pos phase/1
  eta LF/1 -> y-position/1, x-position/1
  psi wave/1 -> cos/1, sin/1
  Product6/1 -> Sum5/2
  y-position/1 -> Product2/2
  x-position/1 -> Product6/2
  cos/1 -> Product6/1
  sin/1 -> Product2/1
  Product2/1 -> Sum5/1
  Sum5/1 -> Product7/1

== system mssSimulink/Modelling/Environmental Loads/Utilities/RAO tables ==
  psi_r : Inport
  omega : Inport  Port=2
  U : Inport  Port=3
  Abs : Abs
  Amplitude table lookup1 : Lookup_n-D  NumberOfTableDimensions=3  BreakpointsForDimension1=RAO_Freq  BreakpointsForDimension2=RAO_Dir  BreakpointsForDimension3=RAO_Vel  Table=RAO_Amp{1}  DiagnosticForOutOfRangeInput=Warning  InternalRulePriority=Speed  RndMeth=Simplest
      settings: InputPortMap=u0,u1,u2
  Amplitude table lookup2 : Lookup_n-D  NumberOfTableDimensions=3  BreakpointsForDimension1=RAO_Freq  BreakpointsForDimension2=RAO_Dir  BreakpointsForDimension3=RAO_Vel  Table=RAO_Amp{2}  InternalRulePriority=Speed  RndMeth=Simplest
      settings: InputPortMap=u0,u1,u2
  Amplitude table lookup3 : Lookup_n-D  NumberOfTableDimensions=3  BreakpointsForDimension1=RAO_Freq  BreakpointsForDimension2=RAO_Dir  BreakpointsForDimension3=RAO_Vel  Table=RAO_Amp{3}  InternalRulePriority=Speed  RndMeth=Simplest
      settings: InputPortMap=u0,u1,u2
  Amplitude table lookup4 : Lookup_n-D  NumberOfTableDimensions=3  BreakpointsForDimension1=RAO_Freq  BreakpointsForDimension2=RAO_Dir  BreakpointsForDimension3=RAO_Vel  Table=RAO_Amp{4}  InternalRulePriority=Speed  RndMeth=Simplest
      settings: InputPortMap=u0,u1,u2
  Amplitude table lookup5 : Lookup_n-D  NumberOfTableDimensions=3  BreakpointsForDimension1=RAO_Freq  BreakpointsForDimension2=RAO_Dir  BreakpointsForDimension3=RAO_Vel  Table=RAO_Amp {5}  InternalRulePriority=Speed  RndMeth=Simplest
      settings: InputPortMap=u0,u1,u2
  Amplitude table lookup6 : Lookup_n-D  NumberOfTableDimensions=3  BreakpointsForDimension1=RAO_Freq  BreakpointsForDimension2=RAO_Dir  BreakpointsForDimension3=RAO_Vel  Table=RAO_Amp{6}  InternalRulePriority=Speed  RndMeth=Simplest
      settings: InputPortMap=u0,u1,u2
  Mux1 : Mux  Inputs=6
  Mux2 : Mux  Inputs=6
  Phase table lookup1 : Lookup_n-D  NumberOfTableDimensions=3  BreakpointsForDimension1=RAO_Freq  BreakpointsForDimension2=RAO_Dir  BreakpointsForDimension3=RAO_Vel  Table=RAO_Phase{1}  InternalRulePriority=Speed  RndMeth=Simplest
      settings: InputPortMap=u0,u1,u2
  Phase table lookup2 : Lookup_n-D  NumberOfTableDimensions=3  BreakpointsForDimension1=RAO_Freq  BreakpointsForDimension2=RAO_Dir  BreakpointsForDimension3=RAO_Vel  Table=RAO_Phase{2}  InternalRulePriority=Speed  RndMeth=Simplest
      settings: InputPortMap=u0,u1,u2
  Phase table lookup3 : Lookup_n-D  NumberOfTableDimensions=3  BreakpointsForDimension1=RAO_Freq  BreakpointsForDimension2=RAO_Dir  BreakpointsForDimension3=RAO_Vel  Table=RAO_Phase{3}  InternalRulePriority=Speed  RndMeth=Simplest
      settings: InputPortMap=u0,u1,u2
  Phase table lookup4 : Lookup_n-D  NumberOfTableDimensions=3  BreakpointsForDimension1=RAO_Freq  BreakpointsForDimension2=RAO_Dir  BreakpointsForDimension3=RAO_Vel  Table=RAO_Phase{4}  InternalRulePriority=Speed  RndMeth=Simplest
      settings: InputPortMap=u0,u1,u2
  Phase table lookup5 : Lookup_n-D  NumberOfTableDimensions=3  BreakpointsForDimension1=RAO_Freq  BreakpointsForDimension2=RAO_Dir  BreakpointsForDimension3=RAO_Vel  Table=RAO_Phase{5}  InternalRulePriority=Speed  RndMeth=Simplest
      settings: InputPortMap=u0,u1,u2
  Phase table lookup6 : Lookup_n-D  NumberOfTableDimensions=3  BreakpointsForDimension1=RAO_Freq  BreakpointsForDimension2=RAO_Dir  BreakpointsForDimension3=RAO_Vel  Table=RAO_Phase{6}  InternalRulePriority=Speed  RndMeth=Simplest
      settings: InputPortMap=u0,u1,u2
  Product1 : Product  Inputs=**  SaturateOnIntegerOverflow=on  OutDataTypeStr=Inherit: Same as first input
  Product2 : Product  Inputs=**  SaturateOnIntegerOverflow=on  OutDataTypeStr=Inherit: Same as first input
  Product3 : Product  Inputs=**  SaturateOnIntegerOverflow=on  OutDataTypeStr=Inherit: Same as first input
  Sign : Signum
  "[-inf inf] to [-pi pi]" : $bdroot/Utilities/Math Operations/[-inf inf] to [-pi pi]
  amp : Outport  VectorParamsAs1DForOutWhenUnconnected=off
  phase : Outport  Port=2  VectorParamsAs1DForOutWhenUnconnected=off
  wires:
  Amplitude table lookup1/1 -> Mux1/1
  omega/1 -> Amplitude table lookup1/1, Phase table lookup1/1, Phase table lookup5/1, Phase table lookup6/1, Phase table lookup4/1, Phase table lookup3/1, Phase table lookup2/1, Amplitude table lookup6/1, Amplitude table lookup5/1, Amplitude table lookup4/1, Amplitude table lookup3/1, Amplitude table lookup2/1
  "[-inf inf] to [-pi pi]"/1 -> Abs/1, Sign/1
  Amplitude table lookup3/1 -> Mux1/3
  Amplitude table lookup5/1 -> Mux1/5
  Abs/1 -> Amplitude table lookup1/2, Phase table lookup1/2, Phase table lookup5/2, Phase table lookup6/2, Phase table lookup4/2, Phase table lookup3/2, Phase table lookup2/2, Amplitude table lookup6/2, Amplitude table lookup5/2, Amplitude table lookup4/2, Amplitude table lookup3/2, Amplitude table lookup2/2
  Product1/1 -> Mux1/2
  Amplitude table lookup2/1 -> Product1/2
  Sign/1 -> Product1/1, Product2/1, Product3/1
  Product2/1 -> Mux1/4
  Amplitude table lookup4/1 -> Product2/2
  Product3/1 -> Mux1/6
  Amplitude table lookup6/1 -> Product3/2
  psi_r/1 -> "[-inf inf] to [-pi pi]"/1
  U/1 -> Amplitude table lookup1/3, Amplitude table lookup2/3, Amplitude table lookup3/3, Amplitude table lookup4/3, Amplitude table lookup6/3, Phase table lookup1/3, Phase table lookup2/3, Phase table lookup3/3, Phase table lookup4/3, Phase table lookup6/3, Phase table lookup5/3, Amplitude table lookup5/3
  Mux2/1 -> phase/1
  Phase table lookup1/1 -> Mux2/1
  Phase table lookup2/1 -> Mux2/2
  Phase table lookup3/1 -> Mux2/3
  Phase table lookup4/1 -> Mux2/4
  Phase table lookup5/1 -> Mux2/5
  Phase table lookup6/1 -> Mux2/6
  Mux1/1 -> amp/1

== system mssSimulink/Modelling/Environmental Loads/Utilities/Signal smoothing ==
  Signal in : Inport
  Signal rate : Inport  Port=2
  -1 : Gain  Gain=-1
  Abs : Abs  SaturateOnIntegerOverflow=off
  Constant : Constant  Value=0  OutDataTypeStr=boolean
  MinMax Running Resettable : simulink/Math Operations/MinMax Running Resettable  Function=max  vinit=0.0
  Rate Limiter Dynamic : simulink/Discontinuities/Rate Limiter Dynamic
  Signal out : Outport  VectorParamsAs1DForOutWhenUnconnected=off
  wires:
  MinMax Running Resettable/1 -> -1/1, Rate Limiter Dynamic/1
  Rate Limiter Dynamic/1 -> Signal out/1
  -1/1 -> Rate Limiter Dynamic/3
  Signal in/1 -> Rate Limiter Dynamic/2
  Constant/1 -> MinMax Running Resettable/2
  Signal rate/1 -> Abs/1
  Abs/1 -> MinMax Running Resettable/1

== system mssSimulink/Modelling/Environmental Loads/Utilities/Yaw quantizer ==
  psi LF : Inport
  psi wave : Inport  Port=2
  Backlash : Backlash  BacklashWidth=back
  Quantizer : Quantizer  QuantizationInterval=quant
  Quantizer flag : Constant  Value=quant_flag
  Sum : Sum  Inputs=|-+
  Switch : Switch  Threshold=0.5  SaturateOnIntegerOverflow=off  InputSameDT=off
  psi_r quantized : Outport  VectorParamsAs1DForOutWhenUnconnected=off
  wires:
  Quantizer flag/1 -> Switch/2
  Switch/1 -> Sum/1
  psi wave/1 -> Sum/2
  Sum/1 -> psi_r quantized/1
  psi LF/1 -> Backlash/1, Switch/3
  Backlash/1 -> Quantizer/1
  Quantizer/1 -> Switch/1

== system mssSimulink/Modelling/Kinetics /Support/3 to 6 DOF ==
  In1 : Inport
  Constant : Constant  Value=0
  Mux1 : Mux  Inputs=2
  Selector : Selector  InputPortWidth=4  IndexOptions=Index vector (dialog)  Indices="[1 2  4 4 4 3]"  OutputSizes=1
  Out1 : Outport  VectorParamsAs1DForOutWhenUnconnected=off
  wires:
  Selector/1 -> Out1/1
  In1/1 -> Mux1/1
  Constant/1 -> Mux1/2
  Mux1/1 -> Selector/1

== system mssSimulink/Modelling/Kinetics /Support/4 to 6 DOF ==
  In1 : Inport
  Constant : Constant  Value=0
  Mux1 : Mux  Inputs=2
  Selector : Selector  InputPortWidth=5  IndexOptions=Index vector (dialog)  Indices="[1 2  5 3 5 4]"  OutputSizes=1
  Out1 : Outport  VectorParamsAs1DForOutWhenUnconnected=off
  wires:
  Selector/1 -> Out1/1
  In1/1 -> Mux1/1
  Constant/1 -> Mux1/2
  Mux1/1 -> Selector/1

== system mssSimulink/Modelling/Kinetics /Support/6 DOF Coriolis forces ==
  M : Inport
  nu : Inport  Port=2
  3x3 cross product : Subsystem  mask(CrossProduct){}
      mask help: Calculate the cross product of two 3-by-1 vectors.
      mask Display:
      | text(.5,.5,'Cross\nProduct\nc = axb', ...
      | 	'HorizontalAlignment','Center',...
      | 	'VerticalAlignment','middle')
  3x3 cross product1 : Subsystem  mask(CrossProduct){}
      mask help: Calculate the cross product of two 3-by-1 vectors.
      mask Display:
      | text(.5,.5,'Cross\nProduct\nc = axb', ...
      | 	'HorizontalAlignment','Center',...
      | 	'VerticalAlignment','middle')
  3x3 cross product2 : Subsystem  mask(CrossProduct){}
      mask help: Calculate the cross product of two 3-by-1 vectors.
      mask Display:
      | text(.5,.5,'Cross\nProduct\nc = axb', ...
      | 	'HorizontalAlignment','Center',...
      | 	'VerticalAlignment','middle')
  Gain : Gain  Gain=0.5  SaturateOnIntegerOverflow=on  OutDataTypeStr=Inherit: Same as input  ParamDataTypeStr=Inherit: Same as input
  Gain1 : Gain  Gain=-1  SaturateOnIntegerOverflow=on  OutDataTypeStr=Inherit: Same as input  ParamDataTypeStr=Inherit: Same as input
  Gain2 : Gain  Gain=-1  SaturateOnIntegerOverflow=on  OutDataTypeStr=Inherit: Same as input  ParamDataTypeStr=Inherit: Same as input
  M11 : Selector  NumberOfDimensions=2  InputPortWidth=3  IndexOptions=Index vector (dialog),Index vector (dialog)  Indices=[1 2 3],[1 2 3]  OutputSizes=1
  M12 : Selector  NumberOfDimensions=2  InputPortWidth=3  IndexOptions=Index vector (dialog),Index vector (dialog)  Indices=[1 2 3],[4 5 6]  OutputSizes=1
  M22 : Selector  NumberOfDimensions=2  InputPortWidth=3  IndexOptions=Index vector (dialog),Index vector (dialog)  Indices=[4 5 6],[4 5 6]  OutputSizes=1
  Mux : Mux  Inputs=2
  Product{,1..3} (4 alike) : Product  Multiplication=Matrix(*)  SaturateOnIntegerOverflow=on  OutDataTypeStr=Inherit: Same as first input
  Selector : Selector  InputPortWidth=6  IndexOptions=Index vector (dialog)  Indices=[1 2 3]  OutputSizes=1
  Selector1 : Selector  InputPortWidth=6  IndexOptions=Index vector (dialog)  Indices=[4 5 6]  OutputSizes=1
  Sum{,1..3} (4 alike) : Sum  Inputs=|++  SaturateOnIntegerOverflow=on
  transpose : Math  Operator=transpose  SignedPower=on
  transpose1 : Math  Operator=transpose  SignedPower=on
  C(nu)nu : Outport  VectorParamsAs1DForOutWhenUnconnected=off
  wires:
  M/1 -> Sum/1, transpose/1  "M"
  nu/1 -> Selector1/1, Selector/1
  Mux/1 -> C(nu)nu/1  "C(nu)nu"
  Sum3/1 -> Mux/2
  3x3 cross product2/1(c) -> Sum3/2
  3x3 cross product1/1(c) -> Sum3/1
  Gain2/1 -> 3x3 cross product2/1(a)
  3x3 cross product/1(c) -> Mux/1
  Gain1/1 -> 3x3 cross product/1(a), 3x3 cross product1/1(a)
  Sum2/1 -> Gain2/1  "dT/d(nu2)"
  Product3/1 -> Sum2/2  "M22*nu2"
  M22/1 -> Product3/1
  Product2/1 -> Sum2/1  "M21*nu1"
  transpose1/1 -> Product2/1  "M21=M12'"
  Sum1/1 -> Gain1/1  "dT/d(nu1)"
  Product1/1 -> Sum1/2  "M12*nu2"
  M12/1 -> Product1/1, transpose1/1
  Product/1 -> Sum1/1  "M11*nu1"
  M11/1 -> Product/1
  Selector1/1 -> Product1/2, Product3/2, 3x3 cross product/2(b), 3x3 cross product2/2(b)  "nu2"
  Selector/1 -> Product/2, Product2/2, 3x3 cross product1/2(b)  "nu1"
  Gain/1 -> M11/1, M12/1, M22/1  "1/2 (M+M')"
  Sum/1 -> Gain/1
  transpose/1 -> Sum/2  "M'"

== system mssSimulink/Modelling/Kinetics /Support/M33 to M66 ==
  M33 : Inport
  Product : Product  Inputs=3  Multiplication=Matrix(*)  SaturateOnIntegerOverflow=on  OutDataTypeStr=Inherit: Same as first input
  modes : Constant  Value=[1 0 0; 0 1 0; 0 0 0; 0 0 0; 0 0 0; 0 0 1]
  transpose : Math  Operator=transpose  SignedPower=on
  M66 : Outport  VectorParamsAs1DForOutWhenUnconnected=off
  wires:
  modes/1 -> transpose/1, Product/1
  transpose/1 -> Product/3
  M33/1 -> Product/2
  Product/1 -> M66/1

== system mssSimulink/Modelling/Kinetics /Support/M44 to M66 ==
  M44 : Inport
  Product : Product  Inputs=3  Multiplication=Matrix(*)  SaturateOnIntegerOverflow=on  OutDataTypeStr=Inherit: Same as first input
  modes : Constant  Value=[1 0 0 0; 0 1 0 0; 0 0 0 0; 0 0 1 0; 0 0 0 0; 0 0 0 1]
  transpose : Math  Operator=transpose  SignedPower=on
  M66 : Outport  VectorParamsAs1DForOutWhenUnconnected=off
  wires:
  modes/1 -> transpose/1, Product/1
  transpose/1 -> Product/3
  M44/1 -> Product/2
  Product/1 -> M66/1

== system mssSimulink/Modelling/Propulsion/Actuator Configuration/2 main propellers and 3 tunnel  thrusters ==
  K(n) : Inport
  u : Inport  Port=2
  Mux : Mux  Inputs=5
  "Thruster configuration matrix " : $bdroot/Modelling/Propulsion/Actuator Configuration/Thruster configuration matrix  SystemSampleTime=-1  VariantActivationTime=update diagram  AllowFlexibleInterface=on  Latency=0  AutoFrameSizeCalculation=off
  f=K(n)*u : Product  InputSameDT=on  SaturateOnIntegerOverflow=on  OutDataTypeStr=Inherit: Same as first input
  main propeller : Constant  Value=0
  tau=T(alpha)*f : Product  Multiplication=Matrix(*)  InputSameDT=on  SaturateOnIntegerOverflow=on  OutDataTypeStr=Inherit: Same as first input
  tunnel thruster : Constant  Value=pi/2
  tau : Outport  VectorParamsAs1DForOutWhenUnconnected=off
  wires:
  f=K(n)*u/1 -> tau=T(alpha)*f/2  "Thrust"
  u/1 -> f=K(n)*u/2
  K(n)/1 -> f=K(n)*u/1
  tau=T(alpha)*f/1 -> tau/1  "Generalized force"
  "Thruster configuration matrix "/1 -> tau=T(alpha)*f/1
  tunnel thruster/1 -> Mux/1, Mux/2, Mux/3
  main propeller/1 -> Mux/5, Mux/4
  Mux/1 -> "Thruster configuration matrix "/1

== system mssSimulink/Modelling/Propulsion/Actuator Configuration/2 main propellers, 1 azimuth and 2 tunnel thrusters ==
  alpha : Inport
  K(n) : Inport  Port=2
  u : Inport  Port=3
  Mux : Mux  Inputs=5
  "Thruster configuration matrix " : $bdroot/Modelling/Propulsion/Actuator Configuration/Thruster configuration matrix  SystemSampleTime=-1  VariantActivationTime=update diagram  AllowFlexibleInterface=on  Latency=0  AutoFrameSizeCalculation=off
  f=K(n)*u : Product  InputSameDT=on  SaturateOnIntegerOverflow=on  OutDataTypeStr=Inherit: Same as first input
  main propeller : Constant  Value=0
  tau=T(alpha)*f : Product  Multiplication=Matrix(*)  InputSameDT=on  SaturateOnIntegerOverflow=on  OutDataTypeStr=Inherit: Same as first input
  tunnel thruster : Constant  Value=pi/2
  tau : Outport  VectorParamsAs1DForOutWhenUnconnected=off
  wires:
  f=K(n)*u/1 -> tau=T(alpha)*f/2  "Thrust"
  u/1 -> f=K(n)*u/2
  K(n)/1 -> f=K(n)*u/1
  tau=T(alpha)*f/1 -> tau/1  "Generalized force"
  alpha/1 -> Mux/3
  "Thruster configuration matrix "/1 -> tau=T(alpha)*f/1
  tunnel thruster/1 -> Mux/1, Mux/2
  main propeller/1 -> Mux/5, Mux/4
  Mux/1 -> "Thruster configuration matrix "/1

== system mssSimulink/Modelling/Propulsion/Actuator Configuration/4 azimuth thrusters ==
  alpha : Inport
  K(n) : Inport  Port=2
  u : Inport  Port=3
  "Thruster configuration matrix  " : $bdroot/Modelling/Propulsion/Actuator Configuration/Thruster configuration matrix  SystemSampleTime=-1  VariantActivationTime=update diagram  AllowFlexibleInterface=on  Latency=0  AutoFrameSizeCalculation=off
  f=K(n)*u : Product  InputSameDT=on  SaturateOnIntegerOverflow=on  OutDataTypeStr=Inherit: Same as first input
  tau=T(alpha)*f : Product  Multiplication=Matrix(*)  InputSameDT=on  SaturateOnIntegerOverflow=on  OutDataTypeStr=Inherit: Same as first input
  tau : Outport  VectorParamsAs1DForOutWhenUnconnected=off
  wires:
  f=K(n)*u/1 -> tau=T(alpha)*f/2  "Thrust"
  u/1 -> f=K(n)*u/2
  K(n)/1 -> f=K(n)*u/1
  tau=T(alpha)*f/1 -> tau/1  "Generalized force"
  alpha/1 -> "Thruster configuration matrix  "/1
  "Thruster configuration matrix  "/1 -> tau=T(alpha)*f/1

== system mssSimulink/Modelling/Propulsion/Actuator Configuration/Column vector t ==
  alpha : Inport
  lx : Inport  Port=2
  ly : Inport  Port=3
  "  " : Trigonometry  Operator=cos
  "   " : Trigonometry
  "    " : Product  InputSameDT=on  SaturateOnIntegerOverflow=on  OutDataTypeStr=Inherit: Same as first input
  "       " : Product  InputSameDT=on  SaturateOnIntegerOverflow=on  OutDataTypeStr=Inherit: Same as first input
  Sum : Sum  Inputs=|-+  InputSameDT=on  SaturateOnIntegerOverflow=on  OutDataTypeStr=Inherit: Same as first input
  Thruster column vector : Concatenate  NumInputs=3  Mode=Multidimensional array
  t : Outport  VectorParamsAs1DForOutWhenUnconnected=off
  wires:
  "  "/1 -> Thruster column vector/1, "       "/1
  "   "/1 -> Thruster column vector/2, "    "/1
  alpha/1 -> "  "/1, "   "/1
  Thruster column vector/1 -> t/1
  "       "/1 -> Sum/1
  lx/1 -> "    "/2
  "    "/1 -> Sum/2
  Sum/1 -> Thruster column vector/3
  ly/1 -> "       "/2

== system mssSimulink/Modelling/Propulsion/Actuator Configuration/Thruster configuration matrix ==
  alpha : Inport
  "Column vector t1 " : $bdroot/Modelling/Propulsion/Actuator Configuration/Column vector t  SystemSampleTime=-1  VariantActivationTime=update diagram  AllowFlexibleInterface=on  Latency=0  AutoFrameSizeCalculation=off
  "Column vector t2 " : $bdroot/Modelling/Propulsion/Actuator Configuration/Column vector t  SystemSampleTime=-1  VariantActivationTime=update diagram  AllowFlexibleInterface=on  Latency=0  AutoFrameSizeCalculation=off
  "Column vector t3 " : $bdroot/Modelling/Propulsion/Actuator Configuration/Column vector t  SystemSampleTime=-1  VariantActivationTime=update diagram  AllowFlexibleInterface=on  Latency=0  AutoFrameSizeCalculation=off
  "Column vector t4 " : $bdroot/Modelling/Propulsion/Actuator Configuration/Column vector t  SystemSampleTime=-1  VariantActivationTime=update diagram  AllowFlexibleInterface=on  Latency=0  AutoFrameSizeCalculation=off
  Demux : Demux
      settings: DisplayOption=none
  Thruster Configuration Matrix : Concatenate  NumInputs=4  Mode=Multidimensional array  ConcatenateDimension=2
  lx{1..4} (4 alike) : Constant  Value=0
  ly{1..4} (4 alike) : Constant  Value=0
  T(alpha) : Outport  VectorParamsAs1DForOutWhenUnconnected=off
  wires:
  "Column vector t4 "/1 -> Thruster Configuration Matrix/1
  "Column vector t1 "/1 -> Thruster Configuration Matrix/2
  "Column vector t2 "/1 -> Thruster Configuration Matrix/3
  "Column vector t3 "/1 -> Thruster Configuration Matrix/4
  Demux/1 -> "Column vector t4 "/1
  Demux/2 -> "Column vector t1 "/1
  Demux/3 -> "Column vector t2 "/1
  Demux/4 -> "Column vector t3 "/1
  alpha/1 -> Demux/1
  Thruster Configuration Matrix/1 -> T(alpha)/1
  lx1/1 -> "Column vector t4 "/2
  ly1/1 -> "Column vector t4 "/3
  lx2/1 -> "Column vector t1 "/2
  ly2/1 -> "Column vector t1 "/3
  lx3/1 -> "Column vector t2 "/2
  ly3/1 -> "Column vector t2 "/3
  lx4/1 -> "Column vector t3 "/2
  ly4/1 -> "Column vector t3 "/3

== system mssSimulink/Navigation/Estimators/Kalman filter based autopilot wave filter/0.5*(P+P') ==
  P : Inport
  "    " : Math  Operator=transpose  SignedPower=on
  Gain6 : Gain  Gain=0.5  SaturateOnIntegerOverflow=on  OutDataTypeStr=Inherit: Same as input  ParamDataTypeStr=Inherit: Same as input
  Sum12 : Sum  Inputs=|++  SaturateOnIntegerOverflow=on
  P=P' : Outport  VectorParamsAs1DForOutWhenUnconnected=off
  wires:
  Gain6/1 -> P=P'/1
  Sum12/1 -> Gain6/1
  "    "/1 -> Sum12/1  "P'"
  P/1 -> "    "/1, Sum12/2  "P"

== system mssSimulink/Navigation/Estimators/Kalman filter based autopilot wave filter/matrices ==
  A-matrix : Constant  Value="[0 1 0 0 0;  -w_o^2  -2*w_o*lambda 0 0 0; 0 0 0 1 0; 0 0 0 -1/T -K/T; 0 0 0 0 -1/T_b]"
  EQE'-matrix : Constant  Value=[0 0 0 0 0; 0 q1 0 0 0; 0 0 0 0 0; 0 0 0 q2 0; 0 0 0 0 q3]
  A : Outport  VectorParamsAs1DForOutWhenUnconnected=off
  EQE' : Outport  Port=2  VectorParamsAs1DForOutWhenUnconnected=off
  wires:
  EQE'-matrix/1 -> EQE'/1
  A-matrix/1 -> A/1

== system mssSimulink/Environment/Wind/Wind/Wind gust/Harris spectrum ==
  Freqs : Inport
  u10 : Inport  Port=2
  Constant : Constant  Value=4
  Constant1 : Constant  Value=5/6
  Fcn : Fcn  Expr=u^(8/3)
  Fcn1 : Fcn  Expr=u^2
  Gain : Gain  Gain=2  SaturateOnIntegerOverflow=on  OutDataTypeStr=Inherit: Same as input  ParamDataTypeStr=Inherit: Same as input
  L : Constant  Value=Par_Wind_L
  Math Function : Math  Operator=magnitude^2  SignedPower=on
  Math Function1 : Math  Operator=magnitude^2  SignedPower=on
  Math Function2 : Math  Operator=pow  SignedPower=on
  Product : Product  Inputs=4  SaturateOnIntegerOverflow=on  OutDataTypeStr=Inherit: Same as first input
  Product1 : Product  SaturateOnIntegerOverflow=on  OutDataTypeStr=Inherit: Same as first input
  Product2 : Product  Inputs=/*  SaturateOnIntegerOverflow=on  OutDataTypeStr=Inherit: Same as first input
  Sum : Sum  Inputs=++|  SaturateOnIntegerOverflow=on
  kappa_H : Constant  Value=Par_Wind_kappa_H
  S : Outport  VectorParamsAs1DForOutWhenUnconnected=off
  wires:
  kappa_H/1 -> Product/3
  Fcn/1 -> Product/1
  u10/1 -> Fcn1/1, Fcn/1
  Fcn1/1 -> Gain/1
  Gain/1 -> Sum/2
  Constant/1 -> Product/4
  L/1 -> Product/2, Math Function1/1
  Math Function/1 -> Product1/1
  Math Function1/1 -> Product1/2
  Product1/1 -> Sum/1
  Sum/1 -> Math Function2/1
  Constant1/1 -> Math Function2/2
  Math Function2/1 -> Product2/1
  Product/1 -> Product2/2
  Freqs/1 -> Math Function/1
  Product2/1 -> S/1
